simulink model "Controller_William"  (R2026b)
settings: Solver=ode1  StopTime=10  FixedStep=Ts
model workspace (MAT data in the model file):
  A_lqg = [-73.3248952405  0.18525672161  -14.1652683546  -0.00013106658503  -4.50700887854  -0.000167623137702  13.1129790251  1.55936657632e-05  3.2595316821  3.10094675975e-05  -1.63619475178e-09; -13422.2701762  -4.55947394234  -0.0240785584886  -1.86925945064  -0.0255345986857  -2.37961365156  0.000928894669951  0.212436587994  0.000769406741286  0.422446312642  5.92383248597e-05; 23.1064607802  10.4738258294  -445.632872261  -349.081623351  -141.788505895  -98.7275298994  0  0  0  0  0; 0.447007508465  0  256  0  0  0  0  0  0  0  0; -22.7100281947  0  0  256  0  0  0  0  0  0  0; -1415.62884741  0  0  0  64  0  0  0  0  0  0; 0.825508223185  0.0255314241406  -0.000717326681496  0.0445418076234  -0.000932687180502  0.056965225355  -2228.16437397  -1090.88537234  -553.861361642  -482.078555377  5.56046164256e-07; -1.25465303857e-12  0  0  0  0  0  2048  0  0  0  0; 8.4492557867e-11  0  0  0  0  0  0  1024  0  0  0; -3.5262008556e-11  0  0  0  0  0  0  0  256  0  0; -65680427.6931  -7830.10901534  -105.316157653  -8175.87245061  -111.684668418  -10408.0884493  4.06285191656  929.167134446  3.36527461571  1847.71951706  -0.740900072445]
  Ae = 0
  B_lqg = [-0.0011206954046; -0.203962579156; 3.88355820131e-05; 6.82079328102e-06; -0.000346527529826; -0.0216007819734; 3.8514834749e-16; -1.91444860622e-17; 1.28925411784e-15; -5.38055550475e-16; -1000]
  Be = [1 0]
  C_lqg = [-144427.693107  -7830.10901534  -105.316157653  -8175.87245061  -111.684668418  -10408.0884493  4.06285191656  929.167134446  3.36527461571  1847.71951706  -0.740900072445; 6762.56336412  209.15342656  -5.87634017481  364.886488051  -7.64057338267  466.659126108  -0.103703360892  -43.4124222803  -0.0859295004114  -86.3296752971  0.00455513017759]
  Ce = [1; 0]
  D_lqg = [0; 0]
  De = [1  0; 0  1]
  ISCS_Ad = [1 0 0 0 0 0 0 0 0 0 0 0 ... (144 elements, 12x12)]
  ISCS_Bd = [0.00131225999503; -1.09814507203e-06; -0.00019614934353; 4.00046239138e-08; 1.16959455957e-08; -3.32560996016e-07; -2.0834141004e-05; -1.34719001764e-09; -1.37952257808e-09; -7.06315558733e-10; -9.04083920366e-11; -0.962703722285]
  ISCS_Cd = [1  -58196.0910892  -7821.80386977  -596.862540453  -8099.99414779  -270.001013433  -10370.653893  229.068639186  841.574458807  74.3402132659  1791.09099882  -0.741227498711; 0  4707.0627635  209.125879811  5.94218242363  363.15389046  -3.75718245885  466.092699567  -5.46381887527  -41.3175515922  -1.77675269433  -84.9642226734  0.00455962982605]
  ISCS_Dd = [1.31291612503; -0.0312763121494]
  ISCS_Tu = [2.36716014767  0; 0  -7]
  ISCS_Ty = 139.999695769
  K = [144427.693107  7830.10901534  105.316157653  8175.87245061  111.684668418  10408.0884493  -4.06285191656  -929.167134446  -3.36527461571  -1847.71951706  0.740900072445; -6762.56336412  -209.15342656  5.87634017481  -364.886488051  7.64057338267  -466.659126108  0.103703360892  43.4124222803  0.0859295004114  86.3296752971  -0.00455513017759]
  K1 = 1
  L = [0.0011206954046; 0.203962579156; -3.88355820131e-05; -6.82079328102e-06; 0.000346527529826; 0.0216007819734; -3.8514834749e-16; 1.91444860622e-17; -1.28925411784e-15; 5.38055550475e-16; 1000]
  Ts = 0.001
  qobs = 1e-06
  qw = 100
  r1 = 10
  r2 = 10
settings Model: Creator=williamvandevoir  LastModifiedBy=williamvandevoir

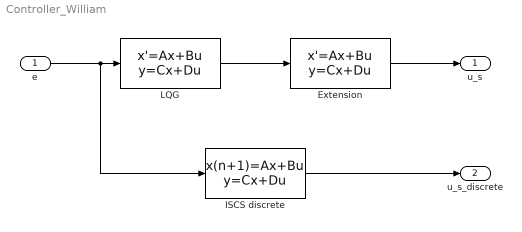
== system Controller_William ==
  e : Inport
  Extension : StateSpace  A=Ae  B=Be  C=Ce  D=De  InitialCondition=0
  ISCS discrete : DiscreteStateSpace  A=ISCS_Ad  B=ISCS_Bd  C=ISCS_Cd  D=ISCS_Dd  InitialCondition=zeros(12,1)  SampleTime=Ts
  LQG : StateSpace  A=A_lqg  B=B_lqg  C=C_lqg  D=D_lqg  InitialCondition=zeros(11,1)
  u_s : Outport
  u_s_discrete : Outport  Port=2
  wires:
  e/1 -> LQG/1, ISCS discrete/1
  LQG/1 -> Extension/1
  Extension/1 -> u_s/1
  ISCS discrete/1 -> u_s_discrete/1
